simulink model "ASM_Traffic"  (R2026a)
settings: Solver=ode1  StartTime=SIM.tstart.v  StopTime=SIM.tend.v  FixedStep=SIM.StepSize.v
PostLoadFcn:
  | if any(exist('dsrtsu_mdlpostloadfcn', 'file') ~= 0), dsrtsu_mdlpostloadfcn('Execute', bdroot); end
  | try, asm_mdl_postloadfcn(bdroot, 'UpdateModel', 3600); catch, disp(lasterr); end,
InitFcn:
  | , if any(exist('rtifpga_mdlclblib', 'file') ~= 0), rtifpga_mdlclblib('Init', bdroot); end,
  | , if any(exist('dsmpb_private', 'file') ~= 0), dsmpb_private('dsmpb_mdlclblib', 'Init', bdroot); end,
model workspace (MAT data in the model file):
  asmReferencePath = [0 0.01 0.02 0.03 0.04 0.05 0.06 0.07 0.08 0.09 0.1 0.11 ... (350007 elements, 50001x7)]
  roadBounds : Simulink.Parameter (value not decoded)
  safetyAxes : Simulink.Parameter (value not decoded)
undefined symbols (not defined in the file): _to_, a0b2, ASM_BrakeHydraulics_DemoSystems, ASM_VehicleDynamics_DemoSystems, b98103fe8ad365046cd0, BrakeCircuit, controllerConfig, CPT, Crankshaft, DiscIntNeverNeededParam, dsmsi, FinalDriveAssembly, MDL, ModeSignals, mu, Pos_BrakePedal_Maneuver, rad, RefSignals, roadFamilyData, roadFamilyId, s_to_rpm, SIM, SoftECU, Suspension, Tire, Transmission
libraries: ASM_Traffic_lib x135, simulink x98, ASM_Utils_lib x77, ASM_VehicleDynamics_lib x70, ASM_Environment_lib x22, dsmpblib x20, dsmsilib x15, MDLD_Utils_lib x10, ASM_BrakeHydraulics_lib x3, sl_discontinuities x2
(part 52 of 65)

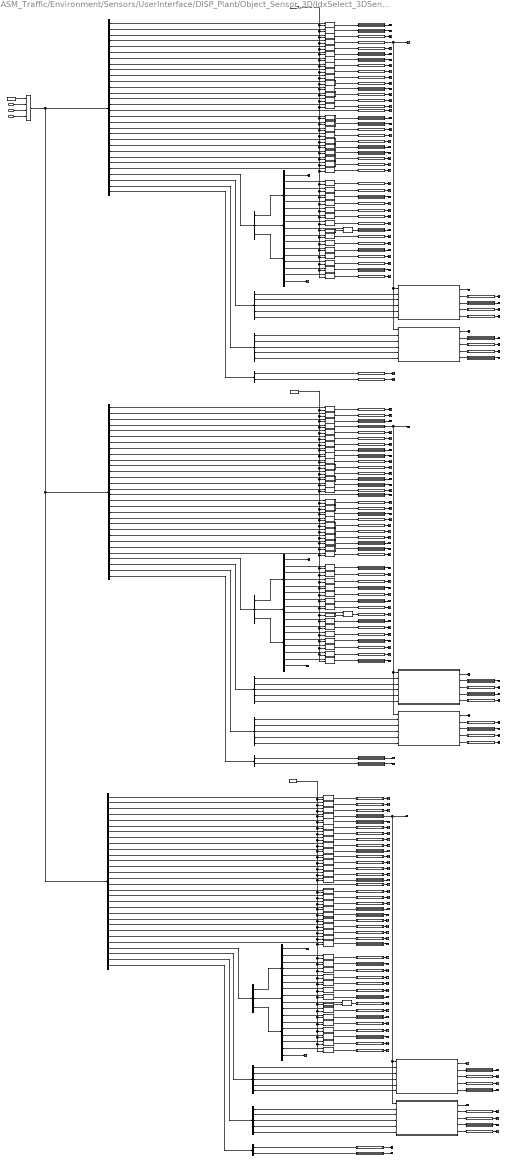
== system ASM_Traffic/Environment/Sensors/UserInterface/DISP_Plant/Object_Sensor_3D/IdxSelect_3DSensor ==
  Sensor_1 : Inport
  Sensor_2 : Inport  Port=2
  Sensor_3 : Inport  Port=3
  Angle_Hor_Object_1[deg] : Subsystem
      mask Display: disp('')
  Angle_Hor_Object_2[deg] : Subsystem
      mask Display: disp('')
  Angle_Hor_Object_3[deg] : Subsystem
      mask Display: disp('')
  Angle_Ver_Object_1[deg] : Subsystem
      mask Display: disp('')
  Angle_Ver_Object_2[deg] : Subsystem
      mask Display: disp('')
  Angle_Ver_Object_3[deg] : Subsystem
      mask Display: disp('')
  Angle_x_Objects_CoorSysE_1[deg] : Subsystem
      mask Display: disp('')
  Angle_x_Objects_CoorSysE_2[deg] : Subsystem
      mask Display: disp('')
  Angle_x_Objects_CoorSysE_3[deg] : Subsystem
      mask Display: disp('')
  Angle_y_Objects_CoorSysE_1[deg] : Subsystem
      mask Display: disp('')
  Angle_y_Objects_CoorSysE_2[deg] : Subsystem
      mask Display: disp('')
  Angle_y_Objects_CoorSysE_3[deg] : Subsystem
      mask Display: disp('')
  Angle_z_Objects_CoorSysE_1[deg] : Subsystem
      mask Display: disp('')
  Angle_z_Objects_CoorSysE_2[deg] : Subsystem
      mask Display: disp('')
  Angle_z_Objects_CoorSysE_3[deg] : Subsystem
      mask Display: disp('')
  Bus Selector : BusSelector  OutputSignals=Object_ID[],ID[],Dist_CoorSys_S[m],Angle_Hor_CoorSys_S[deg],Pos_ObjectPoint_CoorSys_E[x;y;z][m]
  Bus Selector1 : BusSelector  OutputSignals=Info.Flag_Object_In_Scope[0Out|1In],Info.Flag_Sensor_Apex_In_Object[0Out|1In],SensorOutput.Object_Info[-1None|1Fellow|2Static],SensorOutput.Object_ID[],SensorOutput.Object_Type[],SensorOutput.Object_Age[s],SensorOutput.Object_In_Scope_Entry_Number[],SensorOutput.Object_In_Scope_Entry_First[s],SensorOutput.Dist_Object[m],SensorOutput.v_Rel_Object[m|s],SensorOutput.v_Object_CoorSys_S[x;y;z][m|s],SensorOutput.a_Rel_Object[m|s2],SensorOutput.a_Object_CoorSys_S[x;y;z][m|s2],SensorOutput.Angle_Hor_Object[deg],SensorOutput.Angle_Ver_Object[deg],SensorOutput.Pos_Sensor_Apex_E[x;y;z][m],SensorOutput.Pos_Object_NearestPnt_S[x;y;z][m],SensorOutput.Pos_Object_NearestPnt_E[x;y;z][m],SensorOutput.Occlusion_Ratio_Object[-1|0_1],SensorOutput.Flag_NearestPnt_Occluded[-1|0|1],SensorOutput.Pos_NearestSurf_Pnt1_CoorSys_S[x;y;z][m],SensorOutput.Pos_NearestSurf_Pnt2_CoorSys_S[x;y;z][m],SensorOutput.Pos_NearestSurf_Pnt3_CoorSys_S[x;y;z][m],SensorOutput.Pos_NearestSurf_Pnt4_CoorSys_S[x;y;z][m],SensorOutput.NearestSurf_Pnts_Index[],SensorOutput.NearestSurf_Index[],ObjectData,RadarEffects,CustomPoints,SensorTimeStamp
  Bus Selector10 : BusSelector  OutputSignals=Object_Positions,Object_Custom_Values,Object_Properties_Box
  Bus Selector11 : BusSelector  OutputSignals=Object_ID[],ID[],Dist_CoorSys_S[m],Angle_Hor_CoorSys_S[deg],Pos_CoorSys_E[x;y;z][m]
  Bus Selector12 : BusSelector  OutputSignals=Object_ID[],Pos_x_MainPnt_Objects_CoorSysE[m],Pos_y_MainPnt_Objects_CoorSysE[m],Pos_z_MainPnt_Objects_CoorSysE[m],Angle_x_Objects_CoorSysE[deg],Angle_y_Objects_CoorSysE[deg],Angle_z_Objects_CoorSysE[deg]
  Bus Selector13 : BusSelector  OutputSignals=Object_Valid[0|1],CustomValues[]
  Bus Selector14 : BusSelector  OutputSignals=Flag_BoxProperties[0|1],PosVec_x_CenterPnt_Object[m],PosVec_y_CenterPnt_Object[m],PosVec_z_CenterPnt_Object[m],Length_Object[m],Width_Object[m],Height_Object[m],Object_Type[]
  Bus Selector15 : BusSelector  OutputSignals=ObjectSample[s],SensorCalculation[s]
  Bus Selector16 : BusSelector  OutputSignals=Object_Positions,Object_Custom_Values,Object_Properties_Box
  Bus Selector17 : BusSelector  OutputSignals=Object_ID[],ID[],Dist_CoorSys_S[m],Angle_Hor_CoorSys_S[deg],Pos_CoorSys_E[x;y;z][m]
  Bus Selector18 : BusSelector  OutputSignals=Object_ID[],Pos_x_MainPnt_Objects_CoorSysE[m],Pos_y_MainPnt_Objects_CoorSysE[m],Pos_z_MainPnt_Objects_CoorSysE[m],Angle_x_Objects_CoorSysE[deg],Angle_y_Objects_CoorSysE[deg],Angle_z_Objects_CoorSysE[deg]
  Bus Selector19 : BusSelector  OutputSignals=Object_Valid[0|1],CustomValues[]
  Bus Selector2 : BusSelector  OutputSignals=Object_Positions,Object_Custom_Values,Object_Properties_Box
  Bus Selector20 : BusSelector  OutputSignals=Flag_BoxProperties[0|1],PosVec_x_CenterPnt_Object[m],PosVec_y_CenterPnt_Object[m],PosVec_z_CenterPnt_Object[m],Length_Object[m],Width_Object[m],Height_Object[m],Object_Type[]
  Bus Selector21 : BusSelector  OutputSignals=ObjectSample[s],SensorCalculation[s]
  Bus Selector22 : BusSelector  OutputSignals=Object_ID[],ID[],Dist_CoorSys_S[m],Angle_Hor_CoorSys_S[deg],Pos_ObjectPoint_CoorSys_E[x;y;z][m]
  Bus Selector23 : BusSelector  OutputSignals=Info.Flag_Object_In_Scope[0Out|1In],Info.Flag_Sensor_Apex_In_Object[0Out|1In],SensorOutput.Object_Info[-1None|1Fellow|2Static],SensorOutput.Object_ID[],SensorOutput.Object_Type[],SensorOutput.Object_Age[s],SensorOutput.Object_In_Scope_Entry_Number[],SensorOutput.Object_In_Scope_Entry_First[s],SensorOutput.Dist_Object[m],SensorOutput.v_Rel_Object[m|s],SensorOutput.v_Object_CoorSys_S[x;y;z][m|s],SensorOutput.a_Rel_Object[m|s2],SensorOutput.a_Object_CoorSys_S[x;y;z][m|s2],SensorOutput.Angle_Hor_Object[deg],SensorOutput.Angle_Ver_Object[deg],SensorOutput.Pos_Sensor_Apex_E[x;y;z][m],SensorOutput.Pos_Object_NearestPnt_S[x;y;z][m],SensorOutput.Pos_Object_NearestPnt_E[x;y;z][m],SensorOutput.Occlusion_Ratio_Object[-1|0_1],SensorOutput.Flag_NearestPnt_Occluded[-1|0|1],SensorOutput.Pos_NearestSurf_Pnt1_CoorSys_S[x;y;z][m],SensorOutput.Pos_NearestSurf_Pnt2_CoorSys_S[x;y;z][m],SensorOutput.Pos_NearestSurf_Pnt3_CoorSys_S[x;y;z][m],SensorOutput.Pos_NearestSurf_Pnt4_CoorSys_S[x;y;z][m],SensorOutput.NearestSurf_Pnts_Index[],SensorOutput.NearestSurf_Index[],ObjectData,RadarEffects,CustomPoints,SensorTimeStamp
  Bus Selector3 : BusSelector  OutputSignals=Object_ID[],ID[],Dist_CoorSys_S[m],Angle_Hor_CoorSys_S[deg],Pos_CoorSys_E[x;y;z][m]
  Bus Selector4 : BusSelector  OutputSignals=Object_ID[],Pos_x_MainPnt_Objects_CoorSysE[m],Pos_y_MainPnt_Objects_CoorSysE[m],Pos_z_MainPnt_Objects_CoorSysE[m],Angle_x_Objects_CoorSysE[deg],Angle_y_Objects_CoorSysE[deg],Angle_z_Objects_CoorSysE[deg]
  Bus Selector5 : BusSelector  OutputSignals=Object_Valid[0|1],CustomValues[]
  Bus Selector6 : BusSelector  OutputSignals=Flag_BoxProperties[0|1],PosVec_x_CenterPnt_Object[m],PosVec_y_CenterPnt_Object[m],PosVec_z_CenterPnt_Object[m],Length_Object[m],Width_Object[m],Height_Object[m],Object_Type[]
  Bus Selector7 : BusSelector  OutputSignals=ObjectSample[s],SensorCalculation[s]
  Bus Selector8 : BusSelector  OutputSignals=Object_ID[],ID[],Dist_CoorSys_S[m],Angle_Hor_CoorSys_S[deg],Pos_ObjectPoint_CoorSys_E[x;y;z][m]
  Bus Selector9 : BusSelector  OutputSignals=Info.Flag_Object_In_Scope[0Out|1In],Info.Flag_Sensor_Apex_In_Object[0Out|1In],SensorOutput.Object_Info[-1None|1Fellow|2Static],SensorOutput.Object_ID[],SensorOutput.Object_Type[],SensorOutput.Object_Age[s],SensorOutput.Object_In_Scope_Entry_Number[],SensorOutput.Object_In_Scope_Entry_First[s],SensorOutput.Dist_Object[m],SensorOutput.v_Rel_Object[m|s],SensorOutput.v_Object_CoorSys_S[x;y;z][m|s],SensorOutput.a_Rel_Object[m|s2],SensorOutput.a_Object_CoorSys_S[x;y;z][m|s2],SensorOutput.Angle_Hor_Object[deg],SensorOutput.Angle_Ver_Object[deg],SensorOutput.Pos_Sensor_Apex_E[x;y;z][m],SensorOutput.Pos_Object_NearestPnt_S[x;y;z][m],SensorOutput.Pos_Object_NearestPnt_E[x;y;z][m],SensorOutput.Occlusion_Ratio_Object[-1|0_1],SensorOutput.Flag_NearestPnt_Occluded[-1|0|1],SensorOutput.Pos_NearestSurf_Pnt1_CoorSys_S[x;y;z][m],SensorOutput.Pos_NearestSurf_Pnt2_CoorSys_S[x;y;z][m],SensorOutput.Pos_NearestSurf_Pnt3_CoorSys_S[x;y;z][m],SensorOutput.Pos_NearestSurf_Pnt4_CoorSys_S[x;y;z][m],SensorOutput.NearestSurf_Pnts_Index[],SensorOutput.NearestSurf_Index[],ObjectData,RadarEffects,CustomPoints,SensorTimeStamp
  Const_VectorIdx_1[1_15] : Constant
  Const_VectorIdx_2[1_15] : Constant  Value=2
  Const_VectorIdx_3[1_15] : Constant  Value=3
  CustomPoint_Angle_Hor_CoorSys_S_1[deg] : Subsystem
      mask Display: disp('')
  CustomPoint_Angle_Hor_CoorSys_S_2[deg] : Subsystem
      mask Display: disp('')
  CustomPoint_Angle_Hor_CoorSys_S_3[deg] : Subsystem
      mask Display: disp('')
  CustomPoint_Dist_CoorSys_S_1[m] : Subsystem
      mask Display: disp('')
  CustomPoint_Dist_CoorSys_S_2[m] : Subsystem
      mask Display: disp('')
  CustomPoint_Dist_CoorSys_S_3[m] : Subsystem
      mask Display: disp('')
  CustomPoint_ID_1[] : Subsystem
      mask Display: disp('')
  CustomPoint_ID_2[] : Subsystem
      mask Display: disp('')
  CustomPoint_ID_3[] : Subsystem
      mask Display: disp('')
  CustomPoint_Pos_ObjectPoint_CoorSys_E_1[x;y;z][m] : Subsystem
      mask Display: disp('')
  CustomPoint_Pos_ObjectPoint_CoorSys_E_2[x;y;z][m] : Subsystem
      mask Display: disp('')
  CustomPoint_Pos_ObjectPoint_CoorSys_E_3[x;y;z][m] : Subsystem
      mask Display: disp('')
  CustomValues_1[] : Subsystem
      mask Display: disp('')
  CustomValues_2[] : Subsystem
      mask Display: disp('')
  CustomValues_3[] : Subsystem
      mask Display: disp('')
  Dist_Object_1[m] : Subsystem
      mask Display: disp('')
  Dist_Object_2[m] : Subsystem
      mask Display: disp('')
  Dist_Object_3[m] : Subsystem
      mask Display: disp('')
  Flag_BoxProperties_1[0|1] : Subsystem
      mask Display: disp('')
  Flag_BoxProperties_2[0|1] : Subsystem
      mask Display: disp('')
  Flag_BoxProperties_3[0|1] : Subsystem
      mask Display: disp('')
  Flag_NearestPnt_Occluded1[-1|0|1] : Subsystem
      mask Display: disp('')
  Flag_NearestPnt_Occluded2[-1|0|1] : Subsystem
      mask Display: disp('')
  Flag_NearestPnt_Occluded3[-1|0|1] : Subsystem
      mask Display: disp('')
  Flag_Object_In_Scope_1[0Out|1In] : Subsystem
      mask Display: disp('')
  Flag_Object_In_Scope_2[0Out|1In] : Subsystem
      mask Display: disp('')
  Flag_Object_In_Scope_3[0Out|1In] : Subsystem
      mask Display: disp('')
  Flag_Sensor_Apex_In_Object_1[0Out|1In] : Subsystem
      mask Display: disp('')
  Flag_Sensor_Apex_In_Object_2[0Out|1In] : Subsystem
      mask Display: disp('')
  Flag_Sensor_Apex_In_Object_3[0Out|1In] : Subsystem
      mask Display: disp('')
  Height_Object_1[m] : Subsystem
      mask Display: disp('')
  Height_Object_2[m] : Subsystem
      mask Display: disp('')
  Height_Object_3[m] : Subsystem
      mask Display: disp('')
  Length_Object_1[m] : Subsystem
      mask Display: disp('')
  Length_Object_2[m] : Subsystem
      mask Display: disp('')
  Length_Object_3[m] : Subsystem
      mask Display: disp('')
  MaskObjectData_CustomPoints_1 : Subsystem
  MaskObjectData_CustomPoints_2 : Subsystem
  MaskObjectData_CustomPoints_3 : Subsystem
  MaskObjectData_RadarPoints_1 : Subsystem
  MaskObjectData_RadarPoints_2 : Subsystem
  MaskObjectData_RadarPoints_3 : Subsystem
  Multiport Switch : MultiPortSwitch  SaturateOnIntegerOverflow=off  InputSameDT=off
  NearestSurf_Index_1[] : Subsystem
      mask Display: disp('')
  NearestSurf_Index_2[] : Subsystem
      mask Display: disp('')
  NearestSurf_Index_3[] : Subsystem
      mask Display: disp('')
  NearestSurf_Pnts_Index_1[] : Subsystem
      mask Display: disp('')
  NearestSurf_Pnts_Index_2[] : Subsystem
      mask Display: disp('')
  NearestSurf_Pnts_Index_3[] : Subsystem
      mask Display: disp('')
  ObjectSample_1[s] : Subsystem
      mask Display: disp('')
  ObjectSample_2[s] : Subsystem
      mask Display: disp('')
  ObjectSample_3[s] : Subsystem
      mask Display: disp('')
  Object_Age_1[s] : Subsystem
      mask Display: disp('')
  Object_Age_2[s] : Subsystem
      mask Display: disp('')
  Object_Age_3[s] : Subsystem
      mask Display: disp('')
  Object_ID_1[] : Subsystem
      mask Display: disp('')
  Object_ID_2[] : Subsystem
      mask Display: disp('')
  Object_ID_3[] : Subsystem
      mask Display: disp('')
  Object_In_Scope_Entry_First_1[s] : Subsystem
      mask Display: disp('')
  Object_In_Scope_Entry_First_2[s] : Subsystem
      mask Display: disp('')
  Object_In_Scope_Entry_First_3[s] : Subsystem
      mask Display: disp('')
  Object_In_Scope_Entry_Number_1[] : Subsystem
      mask Display: disp('')
  Object_In_Scope_Entry_Number_2[] : Subsystem
      mask Display: disp('')
  Object_In_Scope_Entry_Number_3[] : Subsystem
      mask Display: disp('')
  Object_Info_1[-1None|1Fellow|2Static] : Subsystem
      mask Display: disp('')
  Object_Info_2[-1None|1Fellow|2Static] : Subsystem
      mask Display: disp('')
  Object_Info_3[-1None|1Fellow|2Static] : Subsystem
      mask Display: disp('')
  Object_Type_1[] : Subsystem
      mask Display: disp('')
  Object_Type_2[] : Subsystem
      mask Display: disp('')
  Object_Type_3[] : Subsystem
      mask Display: disp('')
  Object_Valid_1[0|1] : Subsystem
      mask Display: disp('')
  Object_Valid_2[0|1] : Subsystem
      mask Display: disp('')
  Object_Valid_3[0|1] : Subsystem
      mask Display: disp('')
  Occlusion_Ratio_Object1[-1|0_1] : Subsystem
      mask Display: disp('')
  Occlusion_Ratio_Object2[-1|0_1] : Subsystem
      mask Display: disp('')
  Occlusion_Ratio_Object3[-1|0_1] : Subsystem
      mask Display: disp('')
  PosVec_x_CenterPnt_Object_1[m] : Subsystem
      mask Display: disp('')
  PosVec_x_CenterPnt_Object_2[m] : Subsystem
      mask Display: disp('')
  PosVec_x_CenterPnt_Object_3[m] : Subsystem
      mask Display: disp('')
  PosVec_y_CenterPnt_Object_1[m] : Subsystem
      mask Display: disp('')
  PosVec_y_CenterPnt_Object_2[m] : Subsystem
      mask Display: disp('')
  PosVec_y_CenterPnt_Object_3[m] : Subsystem
      mask Display: disp('')
  PosVec_z_CenterPnt_Object_1[m] : Subsystem
      mask Display: disp('')
  PosVec_z_CenterPnt_Object_2[m] : Subsystem
      mask Display: disp('')
  PosVec_z_CenterPnt_Object_3[m] : Subsystem
      mask Display: disp('')
  Pos_NearestSurf_Pnt1_CoorSys_S_1[x;y;z][m] : Subsystem
      mask Display: disp('')
  Pos_NearestSurf_Pnt1_CoorSys_S_2[x;y;z][m] : Subsystem
      mask Display: disp('')
  Pos_NearestSurf_Pnt1_CoorSys_S_3[x;y;z][m] : Subsystem
      mask Display: disp('')
  Pos_NearestSurf_Pnt2_CoorSys_S_1[x;y;z][m] : Subsystem
      mask Display: disp('')
  Pos_NearestSurf_Pnt2_CoorSys_S_2[x;y;z][m] : Subsystem
      mask Display: disp('')
  Pos_NearestSurf_Pnt2_CoorSys_S_3[x;y;z][m] : Subsystem
      mask Display: disp('')
  Pos_NearestSurf_Pnt3_CoorSys_S_1[x;y;z][m] : Subsystem
      mask Display: disp('')
  Pos_NearestSurf_Pnt3_CoorSys_S_2[x;y;z][m] : Subsystem
      mask Display: disp('')
  Pos_NearestSurf_Pnt3_CoorSys_S_3[x;y;z][m] : Subsystem
      mask Display: disp('')
  Pos_NearestSurf_Pnt4_CoorSys_S_1[x;y;z][m] : Subsystem
      mask Display: disp('')
  Pos_NearestSurf_Pnt4_CoorSys_S_2[x;y;z][m] : Subsystem
      mask Display: disp('')
  Pos_NearestSurf_Pnt4_CoorSys_S_3[x;y;z][m] : Subsystem
      mask Display: disp('')
  Pos_Object_NearestPnt_E_1[x;y;z][m] : Subsystem
      mask Display: disp('')
  Pos_Object_NearestPnt_E_2[x;y;z][m] : Subsystem
      mask Display: disp('')
  Pos_Object_NearestPnt_E_3[x;y;z][m] : Subsystem
      mask Display: disp('')
  Pos_Object_NearestPnt_S_1[x;y;z][m] : Subsystem
      mask Display: disp('')
  Pos_Object_NearestPnt_S_2[x;y;z][m] : Subsystem
      mask Display: disp('')
  Pos_Object_NearestPnt_S_3[x;y;z][m] : Subsystem
      mask Display: disp('')
  Pos_Sensor_Apex_E_1[x;y;z][m] : Subsystem
      mask Display: disp('')
  Pos_Sensor_Apex_E_2[x;y;z][m] : Subsystem
      mask Display: disp('')
  Pos_Sensor_Apex_E_3[x;y;z][m] : Subsystem
      mask Display: disp('')
  Pos_x_MainPnt_Objects_CoorSysE_1[m] : Subsystem
      mask Display: disp('')
  Pos_x_MainPnt_Objects_CoorSysE_2[m] : Subsystem
      mask Display: disp('')
  Pos_x_MainPnt_Objects_CoorSysE_3[m] : Subsystem
      mask Display: disp('')
  Pos_y_MainPnt_Objects_CoorSysE_1[m] : Subsystem
      mask Display: disp('')
  Pos_y_MainPnt_Objects_CoorSysE_2[m] : Subsystem
      mask Display: disp('')
  Pos_y_MainPnt_Objects_CoorSysE_3[m] : Subsystem
      mask Display: disp('')
  Pos_z_MainPnt_Objects_CoorSysE_1[m] : Subsystem
      mask Display: disp('')
  Pos_z_MainPnt_Objects_CoorSysE_2[m] : Subsystem
      mask Display: disp('')
  Pos_z_MainPnt_Objects_CoorSysE_3[m] : Subsystem
      mask Display: disp('')
  RadarPoint_Angle_Hor_CoorSys_S_1[deg] : Subsystem
      mask Display: disp('')
  RadarPoint_Angle_Hor_CoorSys_S_2[deg] : Subsystem
      mask Display: disp('')
  RadarPoint_Angle_Hor_CoorSys_S_3[deg] : Subsystem
      mask Display: disp('')
  RadarPoint_Dist_CoorSys_S_1[m] : Subsystem
      mask Display: disp('')
  RadarPoint_Dist_CoorSys_S_2[m] : Subsystem
      mask Display: disp('')
  RadarPoint_Dist_CoorSys_S_3[m] : Subsystem
      mask Display: disp('')
  RadarPoint_ID_1[] : Subsystem
      mask Display: disp('')
  RadarPoint_ID_2[] : Subsystem
      mask Display: disp('')
  RadarPoint_ID_3[] : Subsystem
      mask Display: disp('')
  RadarPoint_Pos_ObjectPoint_CoorSys_E_1[x;y;z][m] : Subsystem
      mask Display: disp('')
  RadarPoint_Pos_ObjectPoint_CoorSys_E_2[x;y;z][m] : Subsystem
      mask Display: disp('')
  RadarPoint_Pos_ObjectPoint_CoorSys_E_3[x;y;z][m] : Subsystem
      mask Display: disp('')
  Selector{1..20,22..44,46..75,77..93} (90 alike) : Selector  InputPortWidth=MDL.Traffic.Sensors.ObjectSensor3D_Calculation.Const_Sensor_Output_Dimension.v  IndexOptions=Index vector (port)  Indices=[1 3]  OutputSizes=1
  Selector21 : Selector  InputPortWidth=MDL.Traffic.Sensors.ObjectSensor3D_Calculation.Const_Sensor_Output_Dimension.v*10  IndexOptions=Starting and ending indices (port)  Indices=[1 3]  OutputSizes=1
  Selector45 : Selector  InputPortWidth=MDL.Traffic.Sensors.ObjectSensor3D_Calculation.Const_Sensor_Output_Dimension.v*10  IndexOptions=Starting and ending indices (port)  Indices=[1 3]  OutputSizes=1
  Selector76 : Selector  InputPortWidth=MDL.Traffic.Sensors.ObjectSensor3D_Calculation.Const_Sensor_Output_Dimension.v*10  IndexOptions=Starting and ending indices (port)  Indices=[1 3]  OutputSizes=1
  SensorCalculation_1[s] : Subsystem
      mask Display: disp('')
  SensorCalculation_2[s] : Subsystem
      mask Display: disp('')
  SensorCalculation_3[s] : Subsystem
      mask Display: disp('')
  Subsystem : Subsystem
  Subsystem1 : Subsystem
  Subsystem10 : Subsystem
  Subsystem11 : Subsystem
  Subsystem12 : Subsystem
  Subsystem13 : Subsystem
  Subsystem14 : Subsystem
  Subsystem15 : Subsystem
  Subsystem16 : Subsystem
  Subsystem17 : Subsystem
  Subsystem18 : Subsystem
  Subsystem19 : Subsystem
  Subsystem2 : Subsystem
  Subsystem20 : Subsystem
  Subsystem21 : Subsystem
  Subsystem22 : Subsystem
  Subsystem23 : Subsystem
  Subsystem24 : Subsystem
  Subsystem25 : Subsystem
  Subsystem26 : Subsystem
  Subsystem27 : Subsystem
  Subsystem28 : Subsystem
  Subsystem29 : Subsystem
  Subsystem3 : Subsystem
  Subsystem4 : Subsystem
  Subsystem5 : Subsystem
  Subsystem6 : Subsystem
  Subsystem7 : Subsystem
  Subsystem8 : Subsystem
  Subsystem9 : Subsystem
  Sw_Sensor_Selector[] : Constant
  Terminator_{1..165} (165 alike) : Terminator
  Width_Object_1[m] : Subsystem
      mask Display: disp('')
  Width_Object_2[m] : Subsystem
      mask Display: disp('')
  Width_Object_3[m] : Subsystem
      mask Display: disp('')
  a_Object_CoorSys_S_1[x;y;z][m|s2] : Subsystem
      mask Display: disp('')
  a_Object_CoorSys_S_2[x;y;z][m|s2] : Subsystem
      mask Display: disp('')
  a_Object_CoorSys_S_3[x;y;z][m|s2] : Subsystem
      mask Display: disp('')
  a_Rel_Object_1[m|s2] : Subsystem
      mask Display: disp('')
  a_Rel_Object_2[m|s2] : Subsystem
      mask Display: disp('')
  a_Rel_Object_3[m|s2] : Subsystem
      mask Display: disp('')
  v_Object_CoorSys_S_1[x;y;z][m|s] : Subsystem
      mask Display: disp('')
  v_Object_CoorSys_S_2[x;y;z][m|s] : Subsystem
      mask Display: disp('')
  v_Object_CoorSys_S_3[x;y;z][m|s] : Subsystem
      mask Display: disp('')
  v_Rel_Object_1[m|s] : Subsystem
      mask Display: disp('')
  v_Rel_Object_2[m|s] : Subsystem
      mask Display: disp('')
  v_Rel_Object_3[m|s] : Subsystem
      mask Display: disp('')
  wires:
  v_Rel_Object_1[m|s]/1(Out1) -> Terminator_10/1
  a_Rel_Object_1[m|s2]/1(Out1) -> Terminator_9/1
  Object_Type_1[]/1(Out1) -> Terminator_8/1
  Object_Info_1[-1None|1Fellow|2Static]/1(Out1) -> Terminator_7/1
  Flag_Sensor_Apex_In_Object_1[0Out|1In]/1(Out1) -> Terminator_5/1
  Flag_Object_In_Scope_1[0Out|1In]/1(Out1) -> Terminator_4/1
  Dist_Object_1[m]/1(Out1) -> Terminator_3/1
  Angle_Ver_Object_1[deg]/1(Out1) -> Terminator_2/1
  Angle_Hor_Object_1[deg]/1(Out1) -> Terminator_1/1
  Selector10/1 -> Angle_Ver_Object_1[deg]/1(In1)
  Selector9/1 -> Angle_Hor_Object_1[deg]/1(In1)
  Selector8/1 -> a_Rel_Object_1[m|s2]/1(In1)
  Selector7/1 -> v_Rel_Object_1[m|s]/1(In1)
  Selector6/1 -> Dist_Object_1[m]/1(In1)
  Selector5/1 -> Object_Type_1[]/1(In1)
  Selector3/1 -> Object_Info_1[-1None|1Fellow|2Static]/1(In1)
  Selector4/1 -> Object_ID_1[]/1(In1)
  Selector2/1 -> Flag_Sensor_Apex_In_Object_1[0Out|1In]/1(In1)
  Selector1/1 -> Flag_Object_In_Scope_1[0Out|1In]/1(In1)
  Const_VectorIdx_1[1_15]/1 -> Selector13/2, Subsystem1/2(Idx), Subsystem2/2(Idx), Subsystem3/2(Idx), Subsystem4/2(Idx), Subsystem5/2(Idx), Subsystem6/2(Idx), Subsystem8/2(Idx), Selector24/2, Selector14/2, Selector15/2, Selector19/2, Selector20/2, Selector29/2, Selector28/2, Selector27/2, Selector26/2, Selector25/2, Selector23/2, Selector22/2, Subsystem9/1(In), Selector18/2, Selector17/2, Selector16/2, Subsystem7/2(Idx), Selector32/2, Selector31/2, Selector10/2, Selector9/2, Selector8/2, Subsystem/2(Idx), Selector7/2, Selector6/2, Selector12/2, Selector11/2, Selector5/2, Selector4/2, Selector3/2, Selector2/2, Selector1/2
  Bus Selector1/15 -> Selector10/1  "<Angle_Ver_Object[deg]>"
  Bus Selector1/14 -> Selector9/1  "<Angle_Hor_Object[deg]>"
  Bus Selector1/12 -> Selector8/1  "<a_Rel_Object[m|s2]>"
  Bus Selector1/10 -> Selector7/1  "<v_Rel_Object[m|s]>"
  Bus Selector1/9 -> Selector6/1  "<Dist_Object[m]>"
  Bus Selector1/5 -> Selector5/1  "<Object_Type[]>"
  Bus Selector1/4 -> Selector4/1  "<Object_ID[]>"
  Bus Selector1/3 -> Selector3/1  "<Object_Info[-1None|1Fellow|2Static]>"
  Bus Selector1/2 -> Selector2/1  "<Flag_Sensor_Apex_In_Object[0Out|1In]>"
  Bus Selector1/1 -> Selector1/1  "<Flag_Object_In_Scope[0Out|1In]>"
  Bus Selector1/19 -> Selector31/1  "<Occlusion_Ratio_Object[-1|0_1]>"
  Bus Selector1/20 -> Selector32/1  "<Flag_NearestPnt_Occluded[-1|0|1]>"
  Selector31/1 -> Occlusion_Ratio_Object1[-1|0_1]/1(In1)
  Selector32/1 -> Flag_NearestPnt_Occluded1[-1|0|1]/1(In1)
  Occlusion_Ratio_Object1[-1|0_1]/1(Out1) -> Terminator_31/1
  Flag_NearestPnt_Occluded1[-1|0|1]/1(Out1) -> Terminator_32/1
  Bus Selector1/28 -> Bus Selector/1  "<RadarEffects>"
  Bus Selector1/27 -> Bus Selector2/1  "<ObjectData>"
  Bus Selector1/6 -> Selector11/1  "<Object_Age[s]>"
  Bus Selector1/7 -> Selector12/1  "<Object_In_Scope_Entry_Number[]>"
  Bus Selector1/8 -> Selector13/1  "<Object_In_Scope_Entry_First[s]>"
  Bus Selector1/26 -> Selector24/1  "<NearestSurf_Index[]>"
  Bus Selector1/29 -> Bus Selector3/1  "<CustomPoints>"
  Selector11/1 -> Object_Age_1[s]/1(In1)
  Selector12/1 -> Object_In_Scope_Entry_Number_1[]/1(In1)
  Selector13/1 -> Object_In_Scope_Entry_First_1[s]/1(In1)
  Object_Age_1[s]/1(Out1) -> Terminator_18/1
  Object_In_Scope_Entry_Number_1[]/1(Out1) -> Terminator_19/1
  Object_In_Scope_Entry_First_1[s]/1(Out1) -> Terminator_20/1
  Pos_Sensor_Apex_E_1[x;y;z][m]/1(Out1) -> Terminator_21/1
  Pos_Object_NearestPnt_S_1[x;y;z][m]/1(Out1) -> Terminator_22/1
  Pos_Object_NearestPnt_E_1[x;y;z][m]/1(Out1) -> Terminator_23/1
  Pos_NearestSurf_Pnt1_CoorSys_S_1[x;y;z][m]/1(Out1) -> Terminator_24/1
  Pos_NearestSurf_Pnt2_CoorSys_S_1[x;y;z][m]/1(Out1) -> Terminator_25/1
  Pos_NearestSurf_Pnt3_CoorSys_S_1[x;y;z][m]/1(Out1) -> Terminator_26/1
  Pos_NearestSurf_Pnt4_CoorSys_S_1[x;y;z][m]/1(Out1) -> Terminator_27/1
  NearestSurf_Pnts_Index_1[]/1(Out1) -> Terminator_28/1
  Selector24/1 -> NearestSurf_Index_1[]/1(In1)
  NearestSurf_Index_1[]/1(Out1) -> Terminator_29/1
  v_Object_CoorSys_S_1[x;y;z][m|s]/1(Out1) -> Terminator_30/1
  a_Object_CoorSys_S_1[x;y;z][m|s2]/1(Out1) -> Terminator_33/1
  Bus Selector1/11 -> Subsystem/1(U)  "<v_Object_CoorSys_S[x;y;z][m|s]>"
  Subsystem/1(Y) -> v_Object_CoorSys_S_1[x;y;z][m|s]/1(In1)
  Bus Selector1/13 -> Subsystem1/1(U)  "<a_Object_CoorSys_S[x;y;z][m|s2]>"
  Subsystem1/1(Y) -> a_Object_CoorSys_S_1[x;y;z][m|s2]/1(In1)
  Bus Selector1/16 -> Pos_Sensor_Apex_E_1[x;y;z][m]/1(In1)  "<Pos_Sensor_Apex_E[x;y;z][m]>"
  Bus Selector1/17 -> Subsystem2/1(U)  "<Pos_Object_NearestPnt_S[x;y;z][m]>"
  Subsystem2/1(Y) -> Pos_Object_NearestPnt_S_1[x;y;z][m]/1(In1)
  Bus Selector1/18 -> Subsystem3/1(U)  "<Pos_Object_NearestPnt_E[x;y;z][m]>"
  Subsystem3/1(Y) -> Pos_Object_NearestPnt_E_1[x;y;z][m]/1(In1)
  Subsystem4/1(Y) -> Pos_NearestSurf_Pnt1_CoorSys_S_1[x;y;z][m]/1(In1)
  Subsystem5/1(Y) -> Pos_NearestSurf_Pnt2_CoorSys_S_1[x;y;z][m]/1(In1)
  Bus Selector1/25 -> Subsystem7/1(U)  "<NearestSurf_Pnts_Index[]>"
  Subsystem7/1(Y) -> NearestSurf_Pnts_Index_1[]/1(In1)
  Bus Selector1/24 -> Subsystem8/1(U)  "<Pos_NearestSurf_Pnt4_CoorSys_S[x;y;z][m]>"
  Subsystem8/1(Y) -> Pos_NearestSurf_Pnt4_CoorSys_S_1[x;y;z][m]/1(In1)
  Subsystem6/1(Y) -> Pos_NearestSurf_Pnt3_CoorSys_S_1[x;y;z][m]/1(In1)
  Bus Selector1/21 -> Subsystem4/1(U)  "<Pos_NearestSurf_Pnt1_CoorSys_S[x;y;z][m]>"
  Bus Selector1/22 -> Subsystem5/1(U)  "<Pos_NearestSurf_Pnt2_CoorSys_S[x;y;z][m]>"
  Bus Selector1/23 -> Subsystem6/1(U)  "<Pos_NearestSurf_Pnt3_CoorSys_S[x;y;z][m]>"
  Object_ID_1[]/1(Out1) -> Terminator_6/1, MaskObjectData_RadarPoints_1/1(Object_ID_Expected[]), MaskObjectData_CustomPoints_1/1(Object_ID_Expected[])
  Bus Selector/1 -> MaskObjectData_RadarPoints_1/2(Object_ID[])  "<Object_ID[]>"
  Bus Selector/2 -> MaskObjectData_RadarPoints_1/3(ID[])  "<ID[]>"
  Bus Selector/3 -> MaskObjectData_RadarPoints_1/4(Dist_CoorSys_S[m])  "<Dist_CoorSys_S[m]>"
  Bus Selector/4 -> MaskObjectData_RadarPoints_1/5(Angle_Hor_CoorSys_S[deg])  "<Angle_Hor_CoorSys_S[deg]>"
  Bus Selector/5 -> MaskObjectData_RadarPoints_1/6(Pos_ObjectPoint_CoorSys_E[x;y;z][m])  "<Pos_ObjectPoint_CoorSys_E[x;y;z][m]>"
  MaskObjectData_RadarPoints_1/2(ID_Masked[]) -> RadarPoint_ID_1[]/1(In1)
  MaskObjectData_RadarPoints_1/3(Dist_CoorSys_S_Masked[m]) -> RadarPoint_Dist_CoorSys_S_1[m]/1(In1)
  MaskObjectData_RadarPoints_1/4(Angle_Hor_CoorSys_S_Masked[deg]) -> RadarPoint_Angle_Hor_CoorSys_S_1[deg]/1(In1)
  MaskObjectData_RadarPoints_1/5(Pos_ObjectPoint_CoorSys_E_Masked[x;y;z][m]) -> RadarPoint_Pos_ObjectPoint_CoorSys_E_1[x;y;z][m]/1(In1)
  Bus Selector3/1 -> MaskObjectData_CustomPoints_1/2(Object_ID[])  "<Object_ID[]>"
  Bus Selector3/2 -> MaskObjectData_CustomPoints_1/3(ID[])  "<ID[]>"
  Bus Selector3/3 -> MaskObjectData_CustomPoints_1/4(Dist_CoorSys_S[m])  "<Dist_CoorSys_S[m]>"
  Bus Selector3/4 -> MaskObjectData_CustomPoints_1/5(Angle_Hor_CoorSys_S[deg])  "<Angle_Hor_CoorSys_S[deg]>"
  Bus Selector3/5 -> MaskObjectData_CustomPoints_1/6(Pos_ObjectPoint_CoorSys_E[x;y;z][m])  "<Pos_CoorSys_E[x;y;z][m]>"
  MaskObjectData_CustomPoints_1/5(Pos_ObjectPoint_CoorSys_E_Masked[x;y;z][m]) -> CustomPoint_Pos_ObjectPoint_CoorSys_E_1[x;y;z][m]/1(In1)
  MaskObjectData_CustomPoints_1/4(Angle_Hor_CoorSys_S_Masked[deg]) -> CustomPoint_Angle_Hor_CoorSys_S_1[deg]/1(In1)
  MaskObjectData_CustomPoints_1/3(Dist_CoorSys_S_Masked[m]) -> CustomPoint_Dist_CoorSys_S_1[m]/1(In1)
  MaskObjectData_CustomPoints_1/2(ID_Masked[]) -> CustomPoint_ID_1[]/1(In1)
  Bus Selector2/1 -> Bus Selector4/1  "<Object_Positions>"
  Bus Selector2/2 -> Bus Selector5/1  "<Object_Custom_Values>"
  Bus Selector2/3 -> Bus Selector6/1  "<Object_Properties_Box>"
  Bus Selector4/1 -> Terminator_37/1  "<Object_ID[]>"
  Bus Selector4/2 -> Selector14/1  "<Pos_x_MainPnt_Objects_CoorSysE[m]>"
  Bus Selector4/3 -> Selector15/1  "<Pos_y_MainPnt_Objects_CoorSysE[m]>"
  Bus Selector4/4 -> Selector16/1  "<Pos_z_MainPnt_Objects_CoorSysE[m]>"
  Bus Selector4/5 -> Selector17/1  "<Angle_x_Objects_CoorSysE[deg]>"
  Bus Selector4/6 -> Selector18/1  "<Angle_y_Objects_CoorSysE[deg]>"
  Bus Selector4/7 -> Selector19/1  "<Angle_z_Objects_CoorSysE[deg]>"
  Bus Selector5/1 -> Selector20/1  "<Object_Valid[0|1]>"
  Bus Selector5/2 -> Selector21/1  "<CustomValues[]>"
  Bus Selector6/1 -> Selector22/1  "<Flag_BoxProperties[0|1]>"
  Bus Selector6/2 -> Selector23/1  "<PosVec_x_CenterPnt_Object[m]>"
  Bus Selector6/3 -> Selector25/1  "<PosVec_y_CenterPnt_Object[m]>"
  Bus Selector6/4 -> Selector26/1  "<PosVec_z_CenterPnt_Object[m]>"
  Bus Selector6/5 -> Selector27/1  "<Length_Object[m]>"
  Bus Selector6/6 -> Selector28/1  "<Width_Object[m]>"
  Bus Selector6/7 -> Selector29/1  "<Height_Object[m]>"
  Bus Selector6/8 -> Terminator_53/1  "<Object_Type[]>"
  MaskObjectData_RadarPoints_1/1(Object_ID_Masked[]) -> Terminator_11/1
  RadarPoint_ID_1[]/1(Out1) -> Terminator_12/1
  RadarPoint_Dist_CoorSys_S_1[m]/1(Out1) -> Terminator_13/1
  RadarPoint_Angle_Hor_CoorSys_S_1[deg]/1(Out1) -> Terminator_14/1
  RadarPoint_Pos_ObjectPoint_CoorSys_E_1[x;y;z][m]/1(Out1) -> Terminator_15/1
  MaskObjectData_CustomPoints_1/1(Object_ID_Masked[]) -> Terminator_16/1
  Pos_x_MainPnt_Objects_CoorSysE_1[m]/1(Out1) -> Terminator_38/1
  Pos_y_MainPnt_Objects_CoorSysE_1[m]/1(Out1) -> Terminator_39/1
  Pos_z_MainPnt_Objects_CoorSysE_1[m]/1(Out1) -> Terminator_40/1
  Angle_x_Objects_CoorSysE_1[deg]/1(Out1) -> Terminator_41/1
  Angle_y_Objects_CoorSysE_1[deg]/1(Out1) -> Terminator_42/1
  Angle_z_Objects_CoorSysE_1[deg]/1(Out1) -> Terminator_43/1
  Object_Valid_1[0|1]/1(Out1) -> Terminator_44/1
  CustomValues_1[]/1(Out1) -> Terminator_45/1
  Flag_BoxProperties_1[0|1]/1(Out1) -> Terminator_46/1
  PosVec_x_CenterPnt_Object_1[m]/1(Out1) -> Terminator_47/1
  PosVec_y_CenterPnt_Object_1[m]/1(Out1) -> Terminator_48/1
  PosVec_z_CenterPnt_Object_1[m]/1(Out1) -> Terminator_49/1
  Length_Object_1[m]/1(Out1) -> Terminator_50/1
  Width_Object_1[m]/1(Out1) -> Terminator_51/1
  Height_Object_1[m]/1(Out1) -> Terminator_52/1
  Bus Selector1/30 -> Bus Selector7/1  "<SensorTimeStamp>"
  Bus Selector7/1 -> ObjectSample_1[s]/1(In1)  "<ObjectSample[s]>"
  Bus Selector7/2 -> SensorCalculation_1[s]/1(In1)  "<SensorCalculation[s]>"
  ObjectSample_1[s]/1(Out1) -> Terminator_54/1
  SensorCalculation_1[s]/1(Out1) -> Terminator_55/1
  CustomPoint_Pos_ObjectPoint_CoorSys_E_1[x;y;z][m]/1(Out1) -> Terminator_36/1
  CustomPoint_Angle_Hor_CoorSys_S_1[deg]/1(Out1) -> Terminator_35/1
  CustomPoint_Dist_CoorSys_S_1[m]/1(Out1) -> Terminator_34/1
  CustomPoint_ID_1[]/1(Out1) -> Terminator_17/1
  Selector14/1 -> Pos_x_MainPnt_Objects_CoorSysE_1[m]/1(In1)
  Selector15/1 -> Pos_y_MainPnt_Objects_CoorSysE_1[m]/1(In1)
  Selector16/1 -> Pos_z_MainPnt_Objects_CoorSysE_1[m]/1(In1)
  Selector17/1 -> Angle_x_Objects_CoorSysE_1[deg]/1(In1)
  Selector18/1 -> Angle_y_Objects_CoorSysE_1[deg]/1(In1)
  Selector19/1 -> Angle_z_Objects_CoorSysE_1[deg]/1(In1)
  Selector22/1 -> Flag_BoxProperties_1[0|1]/1(In1)
  Selector23/1 -> PosVec_x_CenterPnt_Object_1[m]/1(In1)
  Selector25/1 -> PosVec_y_CenterPnt_Object_1[m]/1(In1)
  Selector26/1 -> PosVec_z_CenterPnt_Object_1[m]/1(In1)
  Selector27/1 -> Length_Object_1[m]/1(In1)
  Selector28/1 -> Width_Object_1[m]/1(In1)
  Selector29/1 -> Height_Object_1[m]/1(In1)
  Selector20/1 -> Object_Valid_1[0|1]/1(In1)
  Selector21/1 -> CustomValues_1[]/1(In1)
  Subsystem9/1(Out) -> Selector21/2
  Sensor_3/1 -> Multiport Switch/4
  Sensor_2/1 -> Multiport Switch/3
  Sensor_1/1 -> Multiport Switch/2
  Sw_Sensor_Selector[]/1 -> Multiport Switch/1
  PosVec_x_CenterPnt_Object_2[m]/1(Out1) -> Terminator_97/1
  Bus Selector9/18 -> Subsystem13/1(U)  "<Pos_Object_NearestPnt_E[x;y;z][m]>"
  Bus Selector9/23 -> Subsystem16/1(U)  "<Pos_NearestSurf_Pnt3_CoorSys_S[x;y;z][m]>"
  Bus Selector9/22 -> Subsystem15/1(U)  "<Pos_NearestSurf_Pnt2_CoorSys_S[x;y;z][m]>"
  Subsystem18/1(Y) -> Pos_NearestSurf_Pnt4_CoorSys_S_2[x;y;z][m]/1(In1)
  Bus Selector9/21 -> Subsystem14/1(U)  "<Pos_NearestSurf_Pnt1_CoorSys_S[x;y;z][m]>"
  Bus Selector9/11 -> Subsystem10/1(U)  "<v_Object_CoorSys_S[x;y;z][m|s]>"
  Pos_NearestSurf_Pnt3_CoorSys_S_2[x;y;z][m]/1(Out1) -> Terminator_74/1
  Subsystem15/1(Y) -> Pos_NearestSurf_Pnt2_CoorSys_S_2[x;y;z][m]/1(In1)
  Subsystem16/1(Y) -> Pos_NearestSurf_Pnt3_CoorSys_S_2[x;y;z][m]/1(In1)
  Object_ID_2[]/1(Out1) -> Terminator_107/1, MaskObjectData_RadarPoints_2/1(Object_ID_Expected[]), MaskObjectData_CustomPoints_2/1(Object_ID_Expected[])
  NearestSurf_Index_2[]/1(Out1) -> Terminator_77/1
  Subsystem17/1(Y) -> NearestSurf_Pnts_Index_2[]/1(In1)
  Object_Age_2[s]/1(Out1) -> Terminator_65/1
  Object_Type_2[]/1(Out1) -> Terminator_109/1
  Subsystem14/1(Y) -> Pos_NearestSurf_Pnt1_CoorSys_S_2[x;y;z][m]/1(In1)
  NearestSurf_Pnts_Index_2[]/1(Out1) -> Terminator_76/1
  Subsystem13/1(Y) -> Pos_Object_NearestPnt_E_2[x;y;z][m]/1(In1)
  Bus Selector9/16 -> Pos_Sensor_Apex_E_2[x;y;z][m]/1(In1)  "<Pos_Sensor_Apex_E[x;y;z][m]>"
  Bus Selector9/25 -> Subsystem17/1(U)  "<NearestSurf_Pnts_Index[]>"
  Bus Selector9/17 -> Subsystem12/1(U)  "<Pos_Object_NearestPnt_S[x;y;z][m]>"
  Bus Selector9/8 -> Selector36/1  "<Object_In_Scope_Entry_First[s]>"
  Flag_NearestPnt_Occluded2[-1|0|1]/1(Out1) -> Terminator_81/1
  v_Object_CoorSys_S_2[x;y;z][m|s]/1(Out1) -> Terminator_79/1
  Selector61/1 -> a_Rel_Object_2[m|s2]/1(In1)
  Bus Selector9/13 -> Subsystem11/1(U)  "<a_Object_CoorSys_S[x;y;z][m|s2]>"
  Subsystem11/1(Y) -> a_Object_CoorSys_S_2[x;y;z][m|s2]/1(In1)
  Selector57/1 -> Object_ID_2[]/1(In1)
  a_Object_CoorSys_S_2[x;y;z][m|s2]/1(Out1) -> Terminator_82/1
  Pos_NearestSurf_Pnt2_CoorSys_S_2[x;y;z][m]/1(Out1) -> Terminator_73/1
  Pos_NearestSurf_Pnt4_CoorSys_S_2[x;y;z][m]/1(Out1) -> Terminator_75/1
  Bus Selector9/4 -> Selector57/1  "<Object_ID[]>"
  Selector33/1 -> Angle_Ver_Object_2[deg]/1(In1)
  Pos_Object_NearestPnt_E_2[x;y;z][m]/1(Out1) -> Terminator_71/1
  Selector36/1 -> Object_In_Scope_Entry_First_2[s]/1(In1)
  Object_In_Scope_Entry_Number_2[]/1(Out1) -> Terminator_66/1
  Selector58/1 -> Object_Type_2[]/1(In1)
  Bus Selector9/27 -> Bus Selector10/1  "<ObjectData>"
  Bus Selector9/20 -> Selector56/1  "<Flag_NearestPnt_Occluded[-1|0|1]>"
  Bus Selector9/1 -> Selector30/1  "<Flag_Object_In_Scope[0Out|1In]>"
  Bus Selector9/14 -> Selector62/1  "<Angle_Hor_Object[deg]>"
  Bus Selector9/7 -> Selector35/1  "<Object_In_Scope_Entry_Number[]>"
  v_Rel_Object_2[m|s]/1(Out1) -> Terminator_57/1
  Bus Selector9/6 -> Selector34/1  "<Object_Age[s]>"
  Dist_Object_2[m]/1(Out1) -> Terminator_78/1
  Bus Selector9/28 -> Bus Selector8/1  "<RadarEffects>"
  Bus Selector9/10 -> Selector60/1  "<v_Rel_Object[m|s]>"
  Bus Selector9/9 -> Selector59/1  "<Dist_Object[m]>"
  Pos_NearestSurf_Pnt1_CoorSys_S_2[x;y;z][m]/1(Out1) -> Terminator_72/1
  Bus Selector9/3 -> Selector54/1  "<Object_Info[-1None|1Fellow|2Static]>"
  Bus Selector9/5 -> Selector58/1  "<Object_Type[]>"
  Subsystem12/1(Y) -> Pos_Object_NearestPnt_S_2[x;y;z][m]/1(In1)
  Bus Selector11/1 -> MaskObjectData_CustomPoints_2/2(Object_ID[])  "<Object_ID[]>"
  Bus Selector9/15 -> Selector33/1  "<Angle_Ver_Object[deg]>"
  Bus Selector9/12 -> Selector61/1  "<a_Rel_Object[m|s2]>"
  Selector35/1 -> Object_In_Scope_Entry_Number_2[]/1(In1)
  Angle_Hor_Object_2[deg]/1(Out1) -> Terminator_56/1
  Selector62/1 -> Angle_Hor_Object_2[deg]/1(In1)
  Selector30/1 -> Flag_Object_In_Scope_2[0Out|1In]/1(In1)
  Bus Selector9/26 -> Selector48/1  "<NearestSurf_Index[]>"
  Selector54/1 -> Object_Info_2[-1None|1Fellow|2Static]/1(In1)
  Angle_Ver_Object_2[deg]/1(Out1) -> Terminator_67/1
  Occlusion_Ratio_Object2[-1|0_1]/1(Out1) -> Terminator_80/1
  a_Rel_Object_2[m|s2]/1(Out1) -> Terminator_110/1
  Object_Info_2[-1None|1Fellow|2Static]/1(Out1) -> Terminator_108/1
  Selector44/1 -> Object_Valid_2[0|1]/1(In1)
  Bus Selector14/4 -> Selector50/1  "<PosVec_z_CenterPnt_Object[m]>"
  Selector59/1 -> Dist_Object_2[m]/1(In1)
  Bus Selector14/1 -> Selector46/1  "<Flag_BoxProperties[0|1]>"
  Selector50/1 -> PosVec_z_CenterPnt_Object_2[m]/1(In1)
  Const_VectorIdx_2[1_15]/1 -> Selector36/2, Subsystem11/2(Idx), Subsystem12/2(Idx), Subsystem13/2(Idx), Subsystem14/2(Idx), Subsystem15/2(Idx), Subsystem16/2(Idx), Subsystem18/2(Idx), Selector48/2, Selector37/2, Selector38/2, Selector42/2, Selector44/2, Selector53/2, Selector52/2, Selector51/2, Selector50/2, Selector49/2, Selector47/2, Selector46/2, Subsystem19/1(In), Selector41/2, Selector40/2, Selector39/2, Subsystem17/2(Idx), Selector56/2, Selector55/2, Selector33/2, Selector62/2, Selector61/2, Subsystem10/2(Idx), Selector60/2, Selector59/2, Selector35/2, Selector34/2, Selector58/2, Selector57/2, Selector54/2, Selector43/2, Selector30/2
  Selector39/1 -> Pos_z_MainPnt_Objects_CoorSysE_2[m]/1(In1)
  Selector45/1 -> CustomValues_2[]/1(In1)
  SensorCalculation_2[s]/1(Out1) -> Terminator_106/1
  RadarPoint_Angle_Hor_CoorSys_S_2[deg]/1(Out1) -> Terminator_61/1
  MaskObjectData_CustomPoints_2/2(ID_Masked[]) -> CustomPoint_ID_2[]/1(In1)
  MaskObjectData_CustomPoints_2/3(Dist_CoorSys_S_Masked[m]) -> CustomPoint_Dist_CoorSys_S_2[m]/1(In1)
  MaskObjectData_CustomPoints_2/4(Angle_Hor_CoorSys_S_Masked[deg]) -> CustomPoint_Angle_Hor_CoorSys_S_2[deg]/1(In1)
  Pos_Sensor_Apex_E_2[x;y;z][m]/1(Out1) -> Terminator_69/1
  MaskObjectData_CustomPoints_2/5(Pos_ObjectPoint_CoorSys_E_Masked[x;y;z][m]) -> CustomPoint_Pos_ObjectPoint_CoorSys_E_2[x;y;z][m]/1(In1)
  MaskObjectData_CustomPoints_2/1(Object_ID_Masked[]) -> Terminator_63/1
  Selector51/1 -> Length_Object_2[m]/1(In1)
  Bus Selector12/1 -> Terminator_86/1  "<Object_ID[]>"
  Pos_x_MainPnt_Objects_CoorSysE_2[m]/1(Out1) -> Terminator_87/1
  Flag_Object_In_Scope_2[0Out|1In]/1(Out1) -> Terminator_89/1
  Selector46/1 -> Flag_BoxProperties_2[0|1]/1(In1)
  Bus Selector12/5 -> Selector40/1  "<Angle_x_Objects_CoorSysE[deg]>"
  RadarPoint_Pos_ObjectPoint_CoorSys_E_2[x;y;z][m]/1(Out1) -> Terminator_62/1
  Bus Selector9/29 -> Bus Selector11/1  "<CustomPoints>"
  MaskObjectData_RadarPoints_2/5(Pos_ObjectPoint_CoorSys_E_Masked[x;y;z][m]) -> RadarPoint_Pos_ObjectPoint_CoorSys_E_2[x;y;z][m]/1(In1)
  MaskObjectData_RadarPoints_2/1(Object_ID_Masked[]) -> Terminator_58/1
  CustomPoint_Pos_ObjectPoint_CoorSys_E_2[x;y;z][m]/1(Out1) -> Terminator_85/1
  CustomPoint_ID_2[]/1(Out1) -> Terminator_64/1
  CustomPoint_Angle_Hor_CoorSys_S_2[deg]/1(Out1) -> Terminator_84/1
  Selector52/1 -> Width_Object_2[m]/1(In1)
  Object_Valid_2[0|1]/1(Out1) -> Terminator_94/1
  Angle_z_Objects_CoorSysE_2[deg]/1(Out1) -> Terminator_93/1
  Bus Selector14/6 -> Selector52/1  "<Width_Object[m]>"
  MaskObjectData_RadarPoints_2/3(Dist_CoorSys_S_Masked[m]) -> RadarPoint_Dist_CoorSys_S_2[m]/1(In1)
  MaskObjectData_RadarPoints_2/4(Angle_Hor_CoorSys_S_Masked[deg]) -> RadarPoint_Angle_Hor_CoorSys_S_2[deg]/1(In1)
  Selector56/1 -> Flag_NearestPnt_Occluded2[-1|0|1]/1(In1)
  Height_Object_2[m]/1(Out1) -> Terminator_103/1
  Selector38/1 -> Pos_y_MainPnt_Objects_CoorSysE_2[m]/1(In1)
  Selector53/1 -> Height_Object_2[m]/1(In1)
  Object_In_Scope_Entry_First_2[s]/1(Out1) -> Terminator_68/1
  Bus Selector9/24 -> Subsystem18/1(U)  "<Pos_NearestSurf_Pnt4_CoorSys_S[x;y;z][m]>"
  Flag_Sensor_Apex_In_Object_2[0Out|1In]/1(Out1) -> Terminator_100/1
  Subsystem19/1(Out) -> Selector45/2
  Bus Selector9/19 -> Selector55/1  "<Occlusion_Ratio_Object[-1|0_1]>"
  Selector48/1 -> NearestSurf_Index_2[]/1(In1)
  Bus Selector10/1 -> Bus Selector12/1  "<Object_Positions>"
  Selector49/1 -> PosVec_y_CenterPnt_Object_2[m]/1(In1)
  Selector41/1 -> Angle_y_Objects_CoorSysE_2[deg]/1(In1)
  Selector40/1 -> Angle_x_Objects_CoorSysE_2[deg]/1(In1)
  ObjectSample_2[s]/1(Out1) -> Terminator_105/1
  Selector42/1 -> Angle_z_Objects_CoorSysE_2[deg]/1(In1)
  Bus Selector14/5 -> Selector51/1  "<Length_Object[m]>"
  Bus Selector8/5 -> MaskObjectData_RadarPoints_2/6(Pos_ObjectPoint_CoorSys_E[x;y;z][m])  "<Pos_ObjectPoint_CoorSys_E[x;y;z][m]>"
  Bus Selector8/3 -> MaskObjectData_RadarPoints_2/4(Dist_CoorSys_S[m])  "<Dist_CoorSys_S[m]>"
  Bus Selector8/1 -> MaskObjectData_RadarPoints_2/2(Object_ID[])  "<Object_ID[]>"
  PosVec_z_CenterPnt_Object_2[m]/1(Out1) -> Terminator_99/1
  Bus Selector10/2 -> Bus Selector13/1  "<Object_Custom_Values>"
  Flag_BoxProperties_2[0|1]/1(Out1) -> Terminator_96/1
  Angle_x_Objects_CoorSysE_2[deg]/1(Out1) -> Terminator_91/1
  Bus Selector8/2 -> MaskObjectData_RadarPoints_2/3(ID[])  "<ID[]>"
  Selector60/1 -> v_Rel_Object_2[m|s]/1(In1)
  Bus Selector12/4 -> Selector39/1  "<Pos_z_MainPnt_Objects_CoorSysE[m]>"
  RadarPoint_ID_2[]/1(Out1) -> Terminator_59/1
  Selector37/1 -> Pos_x_MainPnt_Objects_CoorSysE_2[m]/1(In1)
  Bus Selector11/3 -> MaskObjectData_CustomPoints_2/4(Dist_CoorSys_S[m])  "<Dist_CoorSys_S[m]>"
  Bus Selector11/2 -> MaskObjectData_CustomPoints_2/3(ID[])  "<ID[]>"
  Bus Selector12/7 -> Selector42/1  "<Angle_z_Objects_CoorSysE[deg]>"
  Bus Selector11/5 -> MaskObjectData_CustomPoints_2/6(Pos_ObjectPoint_CoorSys_E[x;y;z][m])  "<Pos_CoorSys_E[x;y;z][m]>"
  RadarPoint_Dist_CoorSys_S_2[m]/1(Out1) -> Terminator_60/1
  Bus Selector11/4 -> MaskObjectData_CustomPoints_2/5(Angle_Hor_CoorSys_S[deg])  "<Angle_Hor_CoorSys_S[deg]>"
  Length_Object_2[m]/1(Out1) -> Terminator_101/1
  Bus Selector14/8 -> Terminator_104/1  "<Object_Type[]>"
  Bus Selector15/2 -> SensorCalculation_2[s]/1(In1)  "<SensorCalculation[s]>"
  Bus Selector9/2 -> Selector43/1  "<Flag_Sensor_Apex_In_Object[0Out|1In]>"
  Bus Selector8/4 -> MaskObjectData_RadarPoints_2/5(Angle_Hor_CoorSys_S[deg])  "<Angle_Hor_CoorSys_S[deg]>"
  Selector34/1 -> Object_Age_2[s]/1(In1)
  Bus Selector9/30 -> Bus Selector15/1  "<SensorTimeStamp>"
  CustomValues_2[]/1(Out1) -> Terminator_95/1
  Bus Selector12/6 -> Selector41/1  "<Angle_y_Objects_CoorSysE[deg]>"
  Selector47/1 -> PosVec_x_CenterPnt_Object_2[m]/1(In1)
  Selector55/1 -> Occlusion_Ratio_Object2[-1|0_1]/1(In1)
  Bus Selector14/2 -> Selector47/1  "<PosVec_x_CenterPnt_Object[m]>"
  PosVec_y_CenterPnt_Object_2[m]/1(Out1) -> Terminator_98/1
  Bus Selector14/3 -> Selector49/1  "<PosVec_y_CenterPnt_Object[m]>"
  Bus Selector14/7 -> Selector53/1  "<Height_Object[m]>"
  Pos_y_MainPnt_Objects_CoorSysE_2[m]/1(Out1) -> Terminator_88/1
  MaskObjectData_RadarPoints_2/2(ID_Masked[]) -> RadarPoint_ID_2[]/1(In1)
  Pos_z_MainPnt_Objects_CoorSysE_2[m]/1(Out1) -> Terminator_90/1
  Bus Selector12/3 -> Selector38/1  "<Pos_y_MainPnt_Objects_CoorSysE[m]>"
  Bus Selector15/1 -> ObjectSample_2[s]/1(In1)  "<ObjectSample[s]>"
  Width_Object_2[m]/1(Out1) -> Terminator_102/1
  CustomPoint_Dist_CoorSys_S_2[m]/1(Out1) -> Terminator_83/1
  Bus Selector12/2 -> Selector37/1  "<Pos_x_MainPnt_Objects_CoorSysE[m]>"
  Selector43/1 -> Flag_Sensor_Apex_In_Object_2[0Out|1In]/1(In1)
  Subsystem10/1(Y) -> v_Object_CoorSys_S_2[x;y;z][m|s]/1(In1)
  Bus Selector13/1 -> Selector44/1  "<Object_Valid[0|1]>"
  Pos_Object_NearestPnt_S_2[x;y;z][m]/1(Out1) -> Terminator_70/1
  Angle_y_Objects_CoorSysE_2[deg]/1(Out1) -> Terminator_92/1
  Bus Selector10/3 -> Bus Selector14/1  "<Object_Properties_Box>"
  Bus Selector13/2 -> Selector45/1  "<CustomValues[]>"
  Multiport Switch/1 -> Bus Selector23/1, Bus Selector9/1, Bus Selector1/1
  Selector70/1 -> Pos_z_MainPnt_Objects_CoorSysE_3[m]/1(In1)
  a_Rel_Object_3[m|s2]/1(Out1) -> Terminator_121/1
  Object_Info_3[-1None|1Fellow|2Static]/1(Out1) -> Terminator_119/1
  Occlusion_Ratio_Object3[-1|0_1]/1(Out1) -> Terminator_146/1
  Selector81/1 -> PosVec_z_CenterPnt_Object_3[m]/1(In1)
  Selector90/1 -> Dist_Object_3[m]/1(In1)
  Bus Selector20/1 -> Selector77/1  "<Flag_BoxProperties[0|1]>"
  Selector66/1 -> Object_In_Scope_Entry_Number_3[]/1(In1)
  Selector85/1 -> Object_Info_3[-1None|1Fellow|2Static]/1(In1)
  Bus Selector23/12 -> Selector92/1  "<a_Rel_Object[m|s2]>"
  Bus Selector23/26 -> Selector79/1  "<NearestSurf_Index[]>"
  Selector63/1 -> Flag_Object_In_Scope_3[0Out|1In]/1(In1)
  Angle_Hor_Object_3[deg]/1(Out1) -> Terminator_122/1
  Angle_Ver_Object_3[deg]/1(Out1) -> Terminator_133/1
  Bus Selector23/9 -> Selector90/1  "<Dist_Object[m]>"
  Bus Selector17/1 -> MaskObjectData_CustomPoints_3/2(Object_ID[])  "<Object_ID[]>"
  Pos_NearestSurf_Pnt1_CoorSys_S_3[x;y;z][m]/1(Out1) -> Terminator_138/1
  Bus Selector23/15 -> Selector64/1  "<Angle_Ver_Object[deg]>"
  Subsystem22/1(Y) -> Pos_Object_NearestPnt_S_3[x;y;z][m]/1(In1)
  Bus Selector23/28 -> Bus Selector22/1  "<RadarEffects>"
  Bus Selector23/6 -> Selector65/1  "<Object_Age[s]>"
  v_Rel_Object_3[m|s]/1(Out1) -> Terminator_123/1
  Bus Selector23/7 -> Selector66/1  "<Object_In_Scope_Entry_Number[]>"
  Bus Selector23/1 -> Selector63/1  "<Flag_Object_In_Scope[0Out|1In]>"
  Bus Selector23/27 -> Bus Selector16/1  "<ObjectData>"
  Selector64/1 -> Angle_Ver_Object_3[deg]/1(In1)
  Bus Selector23/4 -> Selector88/1  "<Object_ID[]>"
  Object_In_Scope_Entry_Number_3[]/1(Out1) -> Terminator_132/1
  Bus Selector23/13 -> Subsystem21/1(U)  "<a_Object_CoorSys_S[x;y;z][m|s2]>"
  Pos_NearestSurf_Pnt2_CoorSys_S_3[x;y;z][m]/1(Out1) -> Terminator_139/1
  Subsystem21/1(Y) -> a_Object_CoorSys_S_3[x;y;z][m|s2]/1(In1)
  a_Object_CoorSys_S_3[x;y;z][m|s2]/1(Out1) -> Terminator_148/1
  v_Object_CoorSys_S_3[x;y;z][m|s]/1(Out1) -> Terminator_145/1
  Bus Selector23/8 -> Selector67/1  "<Object_In_Scope_Entry_First[s]>"
  Bus Selector23/17 -> Subsystem22/1(U)  "<Pos_Object_NearestPnt_S[x;y;z][m]>"
  Bus Selector23/25 -> Subsystem27/1(U)  "<NearestSurf_Pnts_Index[]>"
  Flag_NearestPnt_Occluded3[-1|0|1]/1(Out1) -> Terminator_147/1
  Selector92/1 -> a_Rel_Object_3[m|s2]/1(In1)
  NearestSurf_Index_3[]/1(Out1) -> Terminator_143/1
  Subsystem27/1(Y) -> NearestSurf_Pnts_Index_3[]/1(In1)
  Object_Age_3[s]/1(Out1) -> Terminator_131/1
  NearestSurf_Pnts_Index_3[]/1(Out1) -> Terminator_142/1
  Bus Selector23/16 -> Pos_Sensor_Apex_E_3[x;y;z][m]/1(In1)  "<Pos_Sensor_Apex_E[x;y;z][m]>"
  Subsystem24/1(Y) -> Pos_NearestSurf_Pnt1_CoorSys_S_3[x;y;z][m]/1(In1)
  Selector75/1 -> Object_Valid_3[0|1]/1(In1)
  Object_Type_3[]/1(Out1) -> Terminator_120/1
  Subsystem23/1(Y) -> Pos_Object_NearestPnt_E_3[x;y;z][m]/1(In1)
  Bus Selector20/4 -> Selector81/1  "<PosVec_z_CenterPnt_Object[m]>"
  Bus Selector23/3 -> Selector85/1  "<Object_Info[-1None|1Fellow|2Static]>"
  Subsystem25/1(Y) -> Pos_NearestSurf_Pnt2_CoorSys_S_3[x;y;z][m]/1(In1)
  Pos_NearestSurf_Pnt3_CoorSys_S_3[x;y;z][m]/1(Out1) -> Terminator_140/1
  Subsystem26/1(Y) -> Pos_NearestSurf_Pnt3_CoorSys_S_3[x;y;z][m]/1(In1)
  Selector93/1 -> Angle_Hor_Object_3[deg]/1(In1)
  Subsystem28/1(Y) -> Pos_NearestSurf_Pnt4_CoorSys_S_3[x;y;z][m]/1(In1)
  Bus Selector23/21 -> Subsystem24/1(U)  "<Pos_NearestSurf_Pnt1_CoorSys_S[x;y;z][m]>"
  Bus Selector23/18 -> Subsystem23/1(U)  "<Pos_Object_NearestPnt_E[x;y;z][m]>"
  Bus Selector23/23 -> Subsystem26/1(U)  "<Pos_NearestSurf_Pnt3_CoorSys_S[x;y;z][m]>"
  Flag_Sensor_Apex_In_Object_3[0Out|1In]/1(Out1) -> Terminator_111/1
  Selector84/1 -> Height_Object_3[m]/1(In1)
  Subsystem29/1(Out) -> Selector76/2
  Object_In_Scope_Entry_First_3[s]/1(Out1) -> Terminator_134/1
  Bus Selector23/20 -> Selector87/1  "<Flag_NearestPnt_Occluded[-1|0|1]>"
  Bus Selector23/24 -> Subsystem28/1(U)  "<Pos_NearestSurf_Pnt4_CoorSys_S[x;y;z][m]>"
  Selector69/1 -> Pos_y_MainPnt_Objects_CoorSysE_3[m]/1(In1)
  Selector89/1 -> Object_Type_3[]/1(In1)
  MaskObjectData_RadarPoints_3/4(Angle_Hor_CoorSys_S_Masked[deg]) -> RadarPoint_Angle_Hor_CoorSys_S_3[deg]/1(In1)
  Bus Selector23/10 -> Selector91/1  "<v_Rel_Object[m|s]>"
  Angle_z_Objects_CoorSysE_3[deg]/1(Out1) -> Terminator_159/1
  Bus Selector20/6 -> Selector83/1  "<Width_Object[m]>"
  Selector83/1 -> Width_Object_3[m]/1(In1)
  Object_Valid_3[0|1]/1(Out1) -> Terminator_160/1
  Bus Selector23/14 -> Selector93/1  "<Angle_Hor_Object[deg]>"
  MaskObjectData_RadarPoints_3/5(Pos_ObjectPoint_CoorSys_E_Masked[x;y;z][m]) -> RadarPoint_Pos_ObjectPoint_CoorSys_E_3[x;y;z][m]/1(In1)
  Bus Selector23/29 -> Bus Selector17/1  "<CustomPoints>"
  Height_Object_3[m]/1(Out1) -> Terminator_114/1
  CustomPoint_ID_3[]/1(Out1) -> Terminator_130/1
  CustomPoint_Angle_Hor_CoorSys_S_3[deg]/1(Out1) -> Terminator_150/1
  CustomPoint_Pos_ObjectPoint_CoorSys_E_3[x;y;z][m]/1(Out1) -> Terminator_151/1
  Bus Selector18/5 -> Selector71/1  "<Angle_x_Objects_CoorSysE[deg]>"
  RadarPoint_Pos_ObjectPoint_CoorSys_E_3[x;y;z][m]/1(Out1) -> Terminator_128/1
  Selector77/1 -> Flag_BoxProperties_3[0|1]/1(In1)
  Flag_Object_In_Scope_3[0Out|1In]/1(Out1) -> Terminator_155/1
  Bus Selector18/1 -> Terminator_152/1  "<Object_ID[]>"
  Selector82/1 -> Length_Object_3[m]/1(In1)
  MaskObjectData_CustomPoints_3/1(Object_ID_Masked[]) -> Terminator_129/1
  Const_VectorIdx_3[1_15]/1 -> Selector67/2, Subsystem21/2(Idx), Subsystem22/2(Idx), Subsystem23/2(Idx), Subsystem24/2(Idx), Subsystem25/2(Idx), Subsystem26/2(Idx), Subsystem28/2(Idx), Selector79/2, Selector68/2, Selector69/2, Selector73/2, Selector75/2, Selector84/2, Selector83/2, Selector82/2, Selector81/2, Selector80/2, Selector78/2, Selector77/2, Subsystem29/1(In), Selector72/2, Selector71/2, Selector70/2, Subsystem27/2(Idx), Selector87/2, Selector86/2, Selector64/2, Selector93/2, Selector92/2, Subsystem20/2(Idx), Selector91/2, Selector90/2, Selector66/2, Selector65/2, Selector89/2, Selector88/2, Selector85/2, Selector74/2, Selector63/2
  MaskObjectData_CustomPoints_3/5(Pos_ObjectPoint_CoorSys_E_Masked[x;y;z][m]) -> CustomPoint_Pos_ObjectPoint_CoorSys_E_3[x;y;z][m]/1(In1)
  RadarPoint_Angle_Hor_CoorSys_S_3[deg]/1(Out1) -> Terminator_127/1
  Bus Selector16/3 -> Bus Selector20/1  "<Object_Properties_Box>"
  Bus Selector19/2 -> Selector76/1  "<CustomValues[]>"
  Bus Selector19/1 -> Selector75/1  "<Object_Valid[0|1]>"
  Selector67/1 -> Object_In_Scope_Entry_First_3[s]/1(In1)
  Angle_y_Objects_CoorSysE_3[deg]/1(Out1) -> Terminator_158/1
  MaskObjectData_RadarPoints_3/3(Dist_CoorSys_S_Masked[m]) -> RadarPoint_Dist_CoorSys_S_3[m]/1(In1)
  Bus Selector18/3 -> Selector69/1  "<Pos_y_MainPnt_Objects_CoorSysE[m]>"
  MaskObjectData_RadarPoints_3/2(ID_Masked[]) -> RadarPoint_ID_3[]/1(In1)
  Selector87/1 -> Flag_NearestPnt_Occluded3[-1|0|1]/1(In1)
  MaskObjectData_CustomPoints_3/2(ID_Masked[]) -> CustomPoint_ID_3[]/1(In1)
  Pos_y_MainPnt_Objects_CoorSysE_3[m]/1(Out1) -> Terminator_154/1
  Pos_Object_NearestPnt_E_3[x;y;z][m]/1(Out1) -> Terminator_137/1
  Bus Selector20/7 -> Selector84/1  "<Height_Object[m]>"
  Bus Selector20/3 -> Selector80/1  "<PosVec_y_CenterPnt_Object[m]>"
  SensorCalculation_3[s]/1(Out1) -> Terminator_117/1
  Selector78/1 -> PosVec_x_CenterPnt_Object_3[m]/1(In1)
  CustomValues_3[]/1(Out1) -> Terminator_161/1
  Object_ID_3[]/1(Out1) -> Terminator_118/1, MaskObjectData_RadarPoints_3/1(Object_ID_Expected[]), MaskObjectData_CustomPoints_3/1(Object_ID_Expected[])
  Bus Selector18/6 -> Selector72/1  "<Angle_y_Objects_CoorSysE[deg]>"
  Bus Selector23/5 -> Selector89/1  "<Object_Type[]>"
  PosVec_y_CenterPnt_Object_3[m]/1(Out1) -> Terminator_164/1
  Bus Selector23/2 -> Selector74/1  "<Flag_Sensor_Apex_In_Object[0Out|1In]>"
  Bus Selector21/2 -> SensorCalculation_3[s]/1(In1)  "<SensorCalculation[s]>"
  Bus Selector20/8 -> Terminator_115/1  "<Object_Type[]>"
  Bus Selector23/30 -> Bus Selector21/1  "<SensorTimeStamp>"
  Pos_NearestSurf_Pnt4_CoorSys_S_3[x;y;z][m]/1(Out1) -> Terminator_141/1
  Bus Selector17/4 -> MaskObjectData_CustomPoints_3/5(Angle_Hor_CoorSys_S[deg])  "<Angle_Hor_CoorSys_S[deg]>"
  Length_Object_3[m]/1(Out1) -> Terminator_112/1
  Selector65/1 -> Object_Age_3[s]/1(In1)
  Bus Selector18/2 -> Selector68/1  "<Pos_x_MainPnt_Objects_CoorSysE[m]>"
  RadarPoint_Dist_CoorSys_S_3[m]/1(Out1) -> Terminator_126/1
  MaskObjectData_CustomPoints_3/3(Dist_CoorSys_S_Masked[m]) -> CustomPoint_Dist_CoorSys_S_3[m]/1(In1)
  Bus Selector17/5 -> MaskObjectData_CustomPoints_3/6(Pos_ObjectPoint_CoorSys_E[x;y;z][m])  "<Pos_CoorSys_E[x;y;z][m]>"
  Bus Selector18/7 -> Selector73/1  "<Angle_z_Objects_CoorSysE[deg]>"
  Pos_Object_NearestPnt_S_3[x;y;z][m]/1(Out1) -> Terminator_136/1
  MaskObjectData_RadarPoints_3/1(Object_ID_Masked[]) -> Terminator_124/1
  Bus Selector17/2 -> MaskObjectData_CustomPoints_3/3(ID[])  "<ID[]>"
  Bus Selector23/22 -> Subsystem25/1(U)  "<Pos_NearestSurf_Pnt2_CoorSys_S[x;y;z][m]>"
  CustomPoint_Dist_CoorSys_S_3[m]/1(Out1) -> Terminator_149/1
  Bus Selector18/4 -> Selector70/1  "<Pos_z_MainPnt_Objects_CoorSysE[m]>"
  Selector91/1 -> v_Rel_Object_3[m|s]/1(In1)
  Selector86/1 -> Occlusion_Ratio_Object3[-1|0_1]/1(In1)
  RadarPoint_ID_3[]/1(Out1) -> Terminator_125/1
  PosVec_x_CenterPnt_Object_3[m]/1(Out1) -> Terminator_163/1
  Bus Selector22/2 -> MaskObjectData_RadarPoints_3/3(ID[])  "<ID[]>"
  Subsystem20/1(Y) -> v_Object_CoorSys_S_3[x;y;z][m|s]/1(In1)
  Bus Selector17/3 -> MaskObjectData_CustomPoints_3/4(Dist_CoorSys_S[m])  "<Dist_CoorSys_S[m]>"
  Selector88/1 -> Object_ID_3[]/1(In1)
  Bus Selector16/2 -> Bus Selector19/1  "<Object_Custom_Values>"
  Flag_BoxProperties_3[0|1]/1(Out1) -> Terminator_162/1
  Bus Selector22/1 -> MaskObjectData_RadarPoints_3/2(Object_ID[])  "<Object_ID[]>"
  Pos_x_MainPnt_Objects_CoorSysE_3[m]/1(Out1) -> Terminator_153/1
  PosVec_z_CenterPnt_Object_3[m]/1(Out1) -> Terminator_165/1
  Selector76/1 -> CustomValues_3[]/1(In1)
  Bus Selector23/11 -> Subsystem20/1(U)  "<v_Object_CoorSys_S[x;y;z][m|s]>"
  Selector73/1 -> Angle_z_Objects_CoorSysE_3[deg]/1(In1)
  Bus Selector20/2 -> Selector78/1  "<PosVec_x_CenterPnt_Object[m]>"
  Bus Selector21/1 -> ObjectSample_3[s]/1(In1)  "<ObjectSample[s]>"
  Bus Selector22/3 -> MaskObjectData_RadarPoints_3/4(Dist_CoorSys_S[m])  "<Dist_CoorSys_S[m]>"
  Selector71/1 -> Angle_x_Objects_CoorSysE_3[deg]/1(In1)
  Selector74/1 -> Flag_Sensor_Apex_In_Object_3[0Out|1In]/1(In1)
  Bus Selector22/5 -> MaskObjectData_RadarPoints_3/6(Pos_ObjectPoint_CoorSys_E[x;y;z][m])  "<Pos_ObjectPoint_CoorSys_E[x;y;z][m]>"
  Bus Selector22/4 -> MaskObjectData_RadarPoints_3/5(Angle_Hor_CoorSys_S[deg])  "<Angle_Hor_CoorSys_S[deg]>"
  Bus Selector20/5 -> Selector82/1  "<Length_Object[m]>"
  Selector79/1 -> NearestSurf_Index_3[]/1(In1)
  Dist_Object_3[m]/1(Out1) -> Terminator_144/1
  Pos_z_MainPnt_Objects_CoorSysE_3[m]/1(Out1) -> Terminator_156/1
  Selector80/1 -> PosVec_y_CenterPnt_Object_3[m]/1(In1)
  Width_Object_3[m]/1(Out1) -> Terminator_113/1
  Bus Selector23/19 -> Selector86/1  "<Occlusion_Ratio_Object[-1|0_1]>"
  ObjectSample_3[s]/1(Out1) -> Terminator_116/1
  Selector72/1 -> Angle_y_Objects_CoorSysE_3[deg]/1(In1)
  Selector68/1 -> Pos_x_MainPnt_Objects_CoorSysE_3[m]/1(In1)
  Pos_Sensor_Apex_E_3[x;y;z][m]/1(Out1) -> Terminator_135/1
  Bus Selector16/1 -> Bus Selector18/1  "<Object_Positions>"
  MaskObjectData_CustomPoints_3/4(Angle_Hor_CoorSys_S_Masked[deg]) -> CustomPoint_Angle_Hor_CoorSys_S_3[deg]/1(In1)
  Angle_x_Objects_CoorSysE_3[deg]/1(Out1) -> Terminator_157/1
